simulink model "refroidissement_intelligent_final"  (R2022b)
settings: Solver=ode45  StartTime=0.0  StopTime=1200  MaxStep=1  RelTol=1e-3
model workspace (MAT data in the model file):
  P.Cm = 90000
  P.Cl = 35000
  P.Cr = 18000
  P.Kmc = 550
  P.Kcr = 380
  P.UA0 = 35
  P.Kv = 3
  P.Kfan = 210
  P.Qbase = 1700
  P.Qload = 170
  P.Tref = 90
  P.Ttherm0 = 78
  P.Ttherm1 = 88
  P.Kp = 0.09
  P.Ki = 0.0018
  P.Kaw = 0.1
  P.Pfan = 280
  P.Tm0 = 98
  P.Tl0 = 90
  P.Tr0 = 75
values from neighbouring files (symbols this model uses):
  P = struct("Cm",30000,"Cl",25000,"Cr",10000,"Kmc",2000,"Kcr",2500,"UA0",40,"Kv",2.0,"Kfan",150,                 "Pfan",350,"Qbase",4000,"Qload",20000,"Tref",90,"Ttherm0",75,"Ttherm1",90,                 "Kp",0.2,"Ki",0.005,"Kaw",0.1,"Tm0",80,"Tl0",75,"Tr0",65)    [cosim_webots.m]    (also in initialiser_refroidissement.m = struct('Cm',90000,'Cl',35000,'Cr',18000,   'Kmc',550,'Kcr',3)
settings Model: Creator=zeine  LastModifiedBy=zeine

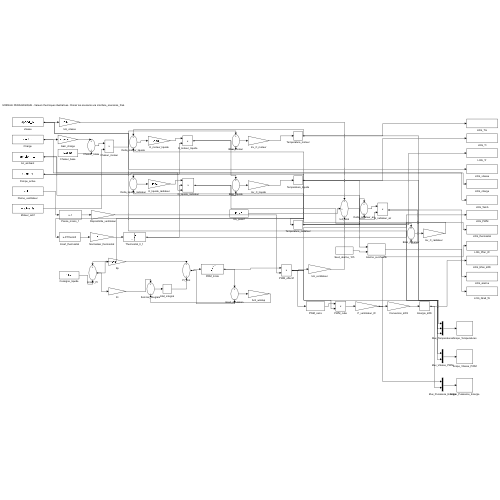
[thumbnail: Simulink's stored preview of the top-level diagram]
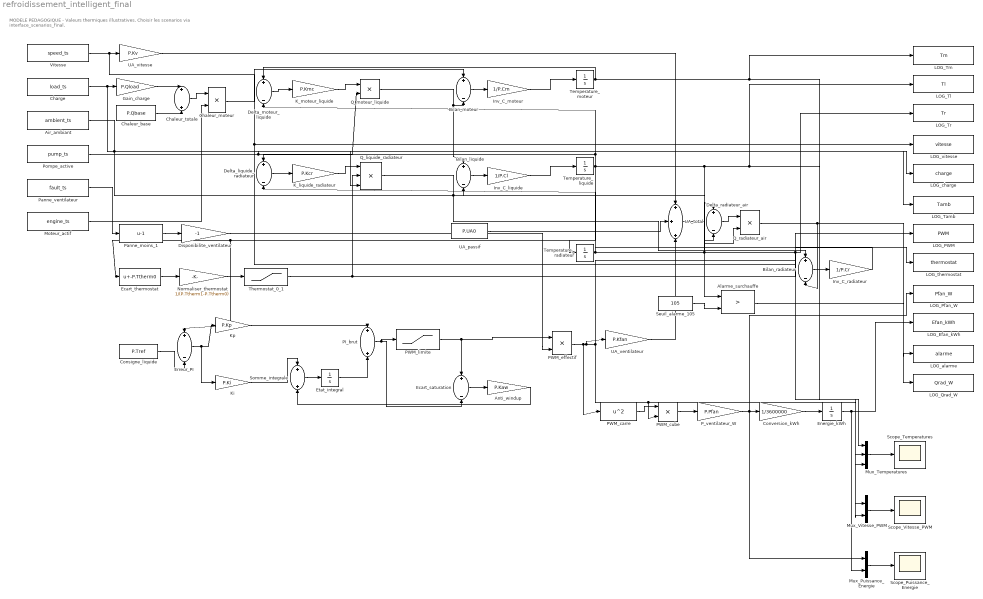
== system refroidissement_intelligent_final ==
  note: MODELE PEDAGOGIQUE - Valeurs thermiques illustratives. Choisir les scenarios via interface_scenarios_final.
  Air_ambiant : FromWorkspace  VariableName=ambient_ts  Interpolate=off  OutputAfterFinalValue=Holding final value
  Alarme_surchauffe : RelationalOperator  Operator=>  OutDataTypeStr=boolean  RndMeth=Simplest  InputSameDT=off
  Anti_windup : Gain  Gain=P.Kaw
  Bilan_liquide : Sum  Inputs=+-
  Bilan_moteur : Sum  Inputs=+-
  Bilan_radiateur : Sum  Inputs=+-
  Chaleur_base : Constant  Value=P.Qbase
  Chaleur_moteur : Product
  Chaleur_totale : Sum
  Charge : FromWorkspace  VariableName=load_ts  Interpolate=off  OutputAfterFinalValue=Holding final value
  Consigne_liquide : Constant  Value=P.Tref
  Conversion_kWh : Gain  Gain=1/3600000
  Delta_liquide_radiateur : Sum  Inputs=+-
  Delta_moteur_liquide : Sum  Inputs=+-
  Delta_radiateur_air : Sum  Inputs=+-
  Disponibilite_ventilateur : Gain  Gain=-1
  Ecart_saturation : Sum  Inputs=+-
  Ecart_thermostat : Bias  Bias=-P.Ttherm0  SaturateOnIntegerOverflow=off
  Energie_kWh : Integrator
  Erreur_PI : Sum  Inputs=+-
  Etat_integral : Integrator
  Gain_charge : Gain  Gain=P.Qload
  Inv_C_liquide : Gain  Gain=1/P.Cl
  Inv_C_moteur : Gain  Gain=1/P.Cm
  Inv_C_radiateur : Gain  Gain=1/P.Cr
  K_liquide_radiateur : Gain  Gain=P.Kcr
  K_moteur_liquide : Gain  Gain=P.Kmc
  Ki : Gain  Gain=P.Ki
  Kp : Gain  Gain=P.Kp
  LOG_Efan_kWh : ToWorkspace  VariableName=Efan_kWh  SaveFormat=Timeseries  SampleTime=-1
  LOG_PWM : ToWorkspace  VariableName=PWM  SaveFormat=Timeseries  SampleTime=-1
  LOG_Pfan_W : ToWorkspace  VariableName=Pfan_W  SaveFormat=Timeseries  SampleTime=-1
  LOG_Qrad_W : ToWorkspace  VariableName=Qrad_W  SaveFormat=Timeseries  SampleTime=-1
  LOG_Tamb : ToWorkspace  VariableName=Tamb  SaveFormat=Timeseries  SampleTime=-1
  LOG_Tl : ToWorkspace  VariableName=Tl  SaveFormat=Timeseries  SampleTime=-1
  LOG_Tm : ToWorkspace  VariableName=Tm  SaveFormat=Timeseries  SampleTime=-1
  LOG_Tr : ToWorkspace  VariableName=Tr  SaveFormat=Timeseries  SampleTime=-1
  LOG_alarme : ToWorkspace  VariableName=alarme  SaveFormat=Timeseries  SampleTime=-1
  LOG_charge : ToWorkspace  VariableName=charge  SaveFormat=Timeseries  SampleTime=-1
  LOG_thermostat : ToWorkspace  VariableName=thermostat  SaveFormat=Timeseries  SampleTime=-1
  LOG_vitesse : ToWorkspace  VariableName=vitesse  SaveFormat=Timeseries  SampleTime=-1
  Moteur_actif : FromWorkspace  VariableName=engine_ts  Interpolate=off  OutputAfterFinalValue=Holding final value
  Mux_Puissance_Energie : Mux  Inputs=2
  Mux_Temperatures : Mux  Inputs=3
  Mux_Vitesse_PWM : Mux  Inputs=2
  Normaliser_thermostat : Gain  Gain=1/(P.Ttherm1-P.Ttherm0)
  PI_brut : Sum
  PWM_carre : Math  Operator=square
  PWM_cube : Product
  PWM_effectif : Product
  PWM_limite : Saturate  UpperLimit=1  LowerLimit=0
  P_ventilateur_W : Gain  Gain=P.Pfan
  Panne_moins_1 : Bias  Bias=-1  SaturateOnIntegerOverflow=off
  Panne_ventilateur : FromWorkspace  VariableName=fault_ts  Interpolate=off  OutputAfterFinalValue=Holding final value
  Pompe_active : FromWorkspace  VariableName=pump_ts  Interpolate=off  OutputAfterFinalValue=Holding final value
  Q_liquide_radiateur : Product  Inputs=***
  Q_moteur_liquide : Product
  Q_radiateur_air : Product
  Scope_Puissance_Energie : Scope
  Scope_Temperatures : Scope
  Scope_Vitesse_PWM : Scope
  Seuil_alarme_105 : Constant  Value=105
  Somme_integrale : Sum
  Temperature_liquide : Integrator  InitialCondition=P.Tl0
  Temperature_moteur : Integrator  InitialCondition=P.Tm0
  Temperature_radiateur : Integrator  InitialCondition=P.Tr0
  Thermostat_0_1 : Saturate  UpperLimit=1  LowerLimit=0
  UA_passif : Constant  Value=P.UA0
  UA_total : Sum  Inputs=+++
  UA_ventilateur : Gain  Gain=P.Kfan
  UA_vitesse : Gain  Gain=P.Kv
  Vitesse : FromWorkspace  VariableName=speed_ts  Interpolate=off  OutputAfterFinalValue=Holding final value
  wires:
  Charge/1 -> Gain_charge/1, LOG_charge/1
  Gain_charge/1 -> Chaleur_totale/1
  Chaleur_base/1 -> Chaleur_totale/2
  Chaleur_totale/1 -> Chaleur_moteur/1
  Moteur_actif/1 -> Chaleur_moteur/2
  Temperature_moteur/1 -> LOG_Tm/1, Mux_Temperatures/1, Delta_moteur_liquide/1
  Temperature_liquide/1 -> Ecart_thermostat/1, Erreur_PI/1, LOG_Tl/1, Mux_Temperatures/2, Alarme_surchauffe/1, Delta_moteur_liquide/2, Delta_liquide_radiateur/1
  Delta_moteur_liquide/1 -> K_moteur_liquide/1
  K_moteur_liquide/1 -> Q_moteur_liquide/1
  Pompe_active/1 -> Q_moteur_liquide/2, Q_liquide_radiateur/3
  Ecart_thermostat/1 -> Normaliser_thermostat/1
  Normaliser_thermostat/1 -> Thermostat_0_1/1
  Temperature_radiateur/1 -> LOG_Tr/1, Mux_Temperatures/3, Delta_radiateur_air/1, Delta_liquide_radiateur/2
  Delta_liquide_radiateur/1 -> K_liquide_radiateur/1
  K_liquide_radiateur/1 -> Q_liquide_radiateur/1
  Thermostat_0_1/1 -> Q_liquide_radiateur/2, LOG_thermostat/1
  Consigne_liquide/1 -> Erreur_PI/2
  Erreur_PI/1 -> Kp/1, Ki/1
  Ki/1 -> Somme_integrale/1
  Anti_windup/1 -> Somme_integrale/2
  Somme_integrale/1 -> Etat_integral/1
  Kp/1 -> PI_brut/1
  Etat_integral/1 -> PI_brut/2
  PI_brut/1 -> PWM_limite/1, Ecart_saturation/2
  PWM_limite/1 -> Ecart_saturation/1, PWM_effectif/1
  Ecart_saturation/1 -> Anti_windup/1
  Panne_ventilateur/1 -> Panne_moins_1/1
  Panne_moins_1/1 -> Disponibilite_ventilateur/1
  Disponibilite_ventilateur/1 -> PWM_effectif/2
  Vitesse/1 -> LOG_vitesse/1, Mux_Vitesse_PWM/1, UA_vitesse/1
  PWM_effectif/1 -> PWM_cube/2, Mux_Vitesse_PWM/2, LOG_PWM/1, UA_ventilateur/1, PWM_carre/1
  UA_vitesse/1 -> UA_total/1
  UA_passif/1 -> UA_total/2
  UA_ventilateur/1 -> UA_total/3
  Air_ambiant/1 -> Delta_radiateur_air/2, LOG_Tamb/1
  Delta_radiateur_air/1 -> Q_radiateur_air/1
  UA_total/1 -> Q_radiateur_air/2
  Chaleur_moteur/1 -> Bilan_moteur/1
  Q_moteur_liquide/1 -> Bilan_moteur/2, Bilan_liquide/1
  Bilan_moteur/1 -> Inv_C_moteur/1
  Inv_C_moteur/1 -> Temperature_moteur/1
  Q_liquide_radiateur/1 -> Bilan_liquide/2, Bilan_radiateur/1
  Bilan_liquide/1 -> Inv_C_liquide/1
  Inv_C_liquide/1 -> Temperature_liquide/1
  Q_radiateur_air/1 -> Bilan_radiateur/2, LOG_Qrad_W/1
  Bilan_radiateur/1 -> Inv_C_radiateur/1
  Inv_C_radiateur/1 -> Temperature_radiateur/1
  PWM_carre/1 -> PWM_cube/1
  PWM_cube/1 -> P_ventilateur_W/1
  P_ventilateur_W/1 -> Conversion_kWh/1, LOG_Pfan_W/1, Mux_Puissance_Energie/1
  Conversion_kWh/1 -> Energie_kWh/1
  Seuil_alarme_105/1 -> Alarme_surchauffe/2
  Energie_kWh/1 -> LOG_Efan_kWh/1, Mux_Puissance_Energie/2
  Alarme_surchauffe/1 -> LOG_alarme/1
  Mux_Temperatures/1 -> Scope_Temperatures/1
  Mux_Vitesse_PWM/1 -> Scope_Vitesse_PWM/1
  Mux_Puissance_Energie/1 -> Scope_Puissance_Energie/1
